simulink model "single_phase_afe_ideal"  (R2026a)
settings: Solver=ode23tb  StopTime=simlength  FixedStep=tc  MaxStep=glb_time.tc
values from neighbouring files (symbols this model uses):
  afe_ctrl = ctrl_afe_setup(glb_time.ts_afe, grid_emu.omega_grid_nom)    [init_model_legacy.m]
  frequency_set = 300    [init_model_legacy.m]
  glb_time = timing_setup(fpwm_afe, trgo_afe, fpwm_inv, trgo_inv, fpwm_single_phase_inv, trgo_single_phase_inv, fpwm_dab, trgo_dab,      fpwm_psfbc, trgo_psfbc, fpwm_isop_rail, trgo_isop_rail, fpwm_cllc, trgo_cllc, t_measure, tc_factor, tc_decimation, delay_pwm, dead_time_afe,      dead_time_inv, dead_time_single_phase_inv, dead_time_dab, dead_time_psfbc, dead_time_isop_rail, dead_time_cllc)    [init_model_legacy.m]
  grid_emu = grid_three_phase_emulator('Dyn11', delta_star, grid_nominal_power, application_voltage, us1, us2, fgrid,                  eq_grid_inductance, eq_grid_resistance, eta, ucc, i1m, p_iron, n1, n2, core_area, core_length, mur,                  up_xi_pu_ref, up_eta_pu_ref, un_xi_pu_ref, un_eta_pu_ref)    [init_model_legacy.m]
  heatsink = liquid_cooled_plate_2kw_setup(weight, no_weight, cp_al, heat_capacity_hs, thermal_conductivity_al,      Rth_switch_HA, Rth_mosfet_HA, Rth_diode_HA, Tambient, DThs_init)    [init_model_legacy.m]
  kepsilon = 2    [init_model_legacy.m]
  omega_set = frequency_set*2*pi    (= 1884.95559215)    [init_model_legacy.m]
  single_phase_inverter_ctrl = ctrl_single_phase_inverter_setup(glb_time.ts_inv, pres_ctrl.omega_set,      dqvector_pi.kp_inv, dqvector_pi.ki_inv, pres_ctrl.kp_rpi, pres_ctrl.ki_rpi, pres_ctrl.delta_rpi)    [init_model_legacy.m]
  Tambient = 40    [init_model_legacy.m]
  time_step_ref_1 = 0.025    [init_model_legacy.m]
  time_step_ref_2 = 0.5    [init_model_legacy.m]
  time_step_ref_3 = 1    [init_model_legacy.m]
  Vdc_nom = 400*1.35    (= 540)    [power_losses_calculation.m]
undefined symbols (not defined in the file or in its folder): delta_fht1, hwdata, igbt, Ld_fht1, magnitude, omega_fht1, ts_inv, Vac_FS, Xbez
libraries: fl_lib x116, nesl_utility x65, phase_shift_filter_ccaller x5, dq_vector_pi x4, igbt_simple_2th_lib x4, linear_double_integrator_observer_ccaller x3, lithium_ion_battery x1, dclink_for_two_levels x1, three_phase_voltage_with_frt_emulator x1, simulink x1, cstblocks_lti x1, single_phase_pwm_modulator x1
(part 4 of 6)

== system single_phase_afe_ideal/single_phase_inverter/single phase inverter control/single_phase_inverter_ctrl/phase generator/FHT-PLL/pll_stageA/filter_and_transformation ==
  ug_a : Inport
  ug_b : Inport  Port=2
  ug_c : Inport  Port=3
  Bus Creator : BusCreator  Inputs=2
  Bus Creator1 : BusCreator  Inputs=3
  Bus Creator2 : BusCreator  Inputs=2
  Bus Creator3 : BusCreator  Inputs=3
  Bus Creator4 : BusCreator  Inputs=3
  FHTalpha : Subsystem
  FHTbeta : Subsystem
  FHTdqPLL : Scope  NumInputPorts=2
      settings: ActiveDisplayYMinimum=-1.5258214459194912  ActiveDisplayYMaximum=1.5258228058860459  DataLoggingVariableName=ScopeData12
  Gain : Gain  Gain=-1/2
  Gain1 : Gain  Gain=-1/2
  Sum : Sum  Inputs=|++
  Sum1 : Sum  Inputs=-+|
  To Workspace1 : ToWorkspace  VariableName=ugd_alpha_sim  SampleTime=-1
      settings: MaxDataPoints=glb_time.Ns_afe
  To Workspace2 : ToWorkspace  VariableName=ugd_beta_sim  SampleTime=-1
      settings: MaxDataPoints=glb_time.Ns_afe
  To Workspace3 : ToWorkspace  VariableName=u_fht_alpha_sim  SampleTime=-1
      settings: MaxDataPoints=glb_time.Ns_afe
  To Workspace4 : ToWorkspace  VariableName=v_fht_alpha_sim  SampleTime=-1
      settings: MaxDataPoints=glb_time.Ns_afe
  To Workspace5 : ToWorkspace  VariableName=u_fhtsr_alpha_sim  SampleTime=-1
      settings: MaxDataPoints=glb_time.Ns_afe
  To Workspace6 : ToWorkspace  VariableName=u_fhtsr_beta_sim  SampleTime=-1
      settings: MaxDataPoints=glb_time.Ns_afe
  To Workspace7 : ToWorkspace  VariableName=u_fht_beta_sim  SampleTime=-1
      settings: MaxDataPoints=glb_time.Ns_afe
  To Workspace8 : ToWorkspace  VariableName=v_fht_beta_sim  SampleTime=-1
      settings: MaxDataPoints=glb_time.Ns_afe
  To Workspace9 : ToWorkspace  VariableName=ugd_abc_grid_sim  SampleTime=-1
      settings: MaxDataPoints=glb_time.Ns_afe
  abc2alphabeta : MATLAB Function  TreatAsAtomicUnit=on
  grid_voltages : Scope  NumInputPorts=3
      settings: ActiveDisplayYMinimum=-1.3620119839906693  ActiveDisplayYMaximum=1.3591613322496414  DataLoggingVariableName=ScopeData13
  ug_alpha : Outport  VectorParamsAs1DForOutWhenUnconnected=off
  ug_beta : Outport  Port=2  VectorParamsAs1DForOutWhenUnconnected=off
  wires:
  ug_b/1 -> Bus Creator3/2, grid_voltages/2, abc2alphabeta/2(b)  "ugd_b"
  ug_c/1 -> Bus Creator3/3, grid_voltages/3, abc2alphabeta/3(c)  "ugd_c"
  ug_a/1 -> Bus Creator3/1, grid_voltages/1, abc2alphabeta/1(a)  "ugd_a"
  abc2alphabeta/1(alpha) -> To Workspace1/1, FHTalpha/1(u), Bus Creator4/1  "u_grid_alpha"
  abc2alphabeta/2(beta) -> FHTbeta/1(u), To Workspace2/1, Bus Creator1/1  "u_grid_beta"
  FHTalpha/1(ud_hat) -> To Workspace3/1, Bus Creator/1, Sum/1  "u_fht_alpha"
  Sum/1 -> Gain/1
  FHTbeta/1(ud_hat) -> Sum1/2, To Workspace7/1, Bus Creator2/1  "u_fht_beta"
  Sum1/1 -> Gain1/1
  Gain1/1 -> Bus Creator1/3, To Workspace6/1, ug_beta/1  "u_fhtsr_beta"
  Gain/1 -> Bus Creator4/3, To Workspace5/1, ug_alpha/1  "u_fhtsr_alpha"
  FHTbeta/2(uq_hat) -> Sum/2, To Workspace8/1, Bus Creator2/2  "v_fht_beta"
  FHTalpha/2(uq_hat) -> Sum1/1, To Workspace4/1, Bus Creator/2  "v_fht_alpha"
  Bus Creator1/1 -> FHTdqPLL/2
  Bus Creator4/1 -> FHTdqPLL/1
  Bus Creator/1 -> Bus Creator4/2  "FHTalpha"
  Bus Creator2/1 -> Bus Creator1/2  "FHTbeta"
  Bus Creator3/1 -> To Workspace9/1

== system single_phase_afe_ideal/single_phase_inverter/single phase inverter control/single_phase_inverter_ctrl/phase generator/FHT-PLL/pll_stageA/sequences ==
  u_grid_alpha : Inport
  u_grid_beta : Inport  Port=2
  phase_angle : Inport  Port=3
  alphabeta2xieta : MATLAB Function  TreatAsAtomicUnit=on
  u_grid_xi : Outport
  u_grid_eta : Outport  Port=2
  wires:
  alphabeta2xieta/1(xi) -> u_grid_xi/1  "u_grid_xi"
  alphabeta2xieta/2(eta) -> u_grid_eta/1  "u_grid_eta"
  u_grid_alpha/1 -> alphabeta2xieta/1(alpha)  "u_grid_alpha"
  u_grid_beta/1 -> alphabeta2xieta/2(beta)  "u_grid_beta"
  phase_angle/1 -> alphabeta2xieta/3(gamma)  "phase_angle"

== system single_phase_afe_ideal/single_phase_inverter/single phase inverter control/single_phase_inverter_ctrl/phase generator/FHT-PLL/pll_stageB/double_integrator_observer ==
  theta : Inport
  Gain : Gain  Gain=afe_ctrl.di_obs.Ldso  Multiplication=Matrix(K*u)
  Gain1 : Gain  Gain=afe_ctrl.di_obs.Adso  Multiplication=Matrix(K*u)
  Gain2 : Gain  Gain=afe_ctrl.di_obs.Cso  Multiplication=Matrix(K*u)
  Selector : Selector  InputPortWidth=2  IndexOptions=Index vector (dialog)  Indices=2  OutputSizes=1
  Sum : Sum  Inputs=-+|
  Sum1 : Sum  Inputs=|++
  Unit Delay : UnitDelay  SampleTime=-1
  bounder1 : MATLAB Function  TreatAsAtomicUnit=on
  bounder2 : MATLAB Function  TreatAsAtomicUnit=on
  omega_hat : Outport
  wires:
  Gain/1 -> Sum1/1
  Selector/1 -> omega_hat/1
  Gain2/1 -> bounder2/1(u)  "theta_hat"
  Gain1/1 -> Sum1/2
  Sum1/1 -> Unit Delay/1
  Sum/1 -> bounder1/1(u)  "e"
  Unit Delay/1 -> Gain1/1, Selector/1, Gain2/1
  theta/1 -> Sum/2  "theta"
  bounder1/1(y) -> Gain/1
  bounder2/1(y) -> Sum/1  "theta_hat_bounded"

== system single_phase_afe_ideal/single_phase_inverter/single phase inverter control/single_phase_inverter_ctrl/single_phase_current_control/dqpi_current_controller/dq_vector_pi_ccaller/Reset ==
  Step : Step  Time=0.05  InitialValue=1  FinalValue=0
  en : Outport
  wires:
  Step/1 -> en/1

== system single_phase_afe_ideal/single_phase_inverter/single phase inverter control/single_phase_inverter_ctrl/single_phase_current_control/dqpi_current_controller/i2alphabeta/first_harmonic_tracker ==
  u : Inport
  Bus Selector : BusSelector  OutputSignals=output_pu_hat,output_pu_hat_dot
  Constant1 : Constant  Value=6
  Constant2 : Constant  Value=glb_time.ts_inv
  Constant3 : Constant  Value=afe_ctrl.fht_grid.omega_fht
  Constant4 : Constant  Value=afe_ctrl.fht_grid.delta_fht
  Constant5 : Constant  Value=afe_ctrl.fht_grid.Ld_fht(1)
  Constant6 : Constant  Value=afe_ctrl.fht_grid.Ld_fht(2)
  Data Type Conversion{1..2,6..9} (6 alike) : DataTypeConversion  OutDataTypeStr=single  SaturateOnIntegerOverflow=off  RndMeth=Floor
  Data Type Conversion10 : DataTypeConversion  OutDataTypeStr=double  SaturateOnIntegerOverflow=off  RndMeth=Floor
  Data Type Conversion3 : DataTypeConversion  OutDataTypeStr=uint8  SaturateOnIntegerOverflow=off  RndMeth=Floor
  Data Type Conversion4 : DataTypeConversion  OutDataTypeStr=double  SaturateOnIntegerOverflow=off  RndMeth=Floor
  Data Type Conversion5 : DataTypeConversion  OutDataTypeStr=uint8  SaturateOnIntegerOverflow=off  RndMeth=Floor
  Gain : Gain  Gain=-1/afe_ctrl.fht_grid.omega_fht
  Step : Step  Time=0.0125  InitialValue=1  FinalValue=0
  first_harmonic_tracker : CCaller  FunctionName=first_harmonic_tracker_process_simulink  PortSpecificationStruct="%)30     .    B \\   8    (     @         %    \"     D    !     0         %  0 \"0    $    _    07)G3F%M90  4&]R=$YA;64 4V-O<&4     26YD97@     5'EP90      4VEZ90      27-';&]B86P   X    P    !@    @    $          4    (     0    ,    !         !   P!O=70 #@   #     &    \"     0         !0    @    !     P    $         $  # &]U=  .    .     8    (    !          %    \"     $    &     0         0  ...(+4988 chars)"
  alpha : Outport
  beta : Outport  Port=2
  wires:
  Data Type Conversion4/1 -> alpha/1
  Data Type Conversion3/1 -> first_harmonic_tracker/1
  Data Type Conversion1/1 -> first_harmonic_tracker/3
  Data Type Conversion2/1 -> first_harmonic_tracker/2
  first_harmonic_tracker/1 -> Bus Selector/1
  Bus Selector/1 -> Data Type Conversion4/1  "<output_pu_hat>"
  Step/1 -> Data Type Conversion3/1
  u/1 -> Data Type Conversion2/1
  Constant2/1 -> Data Type Conversion1/1
  Constant1/1 -> Data Type Conversion5/1
  Data Type Conversion5/1 -> first_harmonic_tracker/8
  Constant3/1 -> Data Type Conversion6/1
  Data Type Conversion6/1 -> first_harmonic_tracker/4
  Constant4/1 -> Data Type Conversion7/1
  Data Type Conversion7/1 -> first_harmonic_tracker/5
  Constant5/1 -> Data Type Conversion8/1
  Data Type Conversion8/1 -> first_harmonic_tracker/6
  Constant6/1 -> Data Type Conversion9/1
  Data Type Conversion9/1 -> first_harmonic_tracker/7
  Bus Selector/2 -> Data Type Conversion10/1  "<output_pu_hat_dot>"
  Data Type Conversion10/1 -> Gain/1
  Gain/1 -> beta/1

== system single_phase_afe_ideal/single_phase_inverter/single phase inverter control/single_phase_inverter_ctrl/single_phase_current_control/dqpi_current_controller/i2alphabeta/phase_shift_method ==
  i_alpha : Inport
  Gain : Gain  Gain=-1
  phase shift filter : phase_shift_filter/phase shift filter  f=frequency_set  scaling_factor=1  ts=glb_time.ts_inv
  i_alpha_phase_shift_m : Outport
  i_beta_phase_shift_m : Outport  Port=2
  wires:
  i_alpha/1 -> phase shift filter/1, i_alpha_phase_shift_m/1
  Gain/1 -> i_beta_phase_shift_m/1  "i_beta_phase_shift_methos"
  phase shift filter/1 -> Gain/1

== system single_phase_afe_ideal/single_phase_inverter/single phase inverter control/single_phase_inverter_ctrl/single_phase_current_control/dqpi_current_controller/i2alphabeta/phase_shift_method_ccaller ==
  i_alpha : Inport
  Gain : Gain  Gain=-1
  phase_shift_filter_ccaller : phase_shift_filter_ccaller/phase_shift_filter_ccaller  freq_m=frequency_set  ts_m=glb_time.ts_inv  scaling_m=1  reset_time_release=0.025  instance=0  tc_m=-1
  i_alpha_phase_shift_m : Outport
  i_beta_phase_shift_m : Outport  Port=2
  wires:
  phase_shift_filter_ccaller/1 -> Gain/1
  Gain/1 -> i_beta_phase_shift_m/1  "i_beta_phase_shift_methos"
  i_alpha/1 -> i_alpha_phase_shift_m/1, phase_shift_filter_ccaller/1

== system single_phase_afe_ideal/single_phase_inverter/single phase inverter control/single_phase_inverter_ctrl/single_phase_current_control/dqpi_current_controller/i2alphabeta/sogi ==
  u : Inport
  Constant2 : Constant  Value=omega_set
  Product : Product
  Product1 : Product
  Sum1 : Sum  Inputs=|+-
  Sum3 : Sum  Inputs=-+|
  integrator_1 : Subsystem
  integrator_2 : Subsystem
  kepsilon : Gain  Gain=kepsilon
  ualpha : Outport
  ubeta : Outport  Port=2
  wires:
  u/1 -> ualpha/1, Sum3/2
  Sum3/1 -> kepsilon/1
  kepsilon/1 -> Sum1/1
  Sum1/1 -> Product/2
  Product/1 -> integrator_1/1(in)
  integrator_1/1(out) -> Product1/2, Sum3/1
  Constant2/1 -> Product/1, Product1/1
  Product1/1 -> integrator_2/1(in)
  integrator_2/1(out) -> ubeta/1, Sum1/2

== system single_phase_afe_ideal/single_phase_inverter/single phase inverter control/single_phase_inverter_ctrl/single_phase_current_control/dqpi_current_controller/i2alphabeta/sogi_ccaller ==
  input : Inport
  Bus Selector : BusSelector  OutputSignals=sogi_flt_output_alpha,sogi_flt_output_beta
  CCaller : CCaller  FunctionName=sogi_flt_process_simulink  PortSpecificationStruct="%)30     .    . P   8    (     @         %    \"     <    !     0         %  0 \"0    $    _    07)G3F%M90  4&]R=$YA;64 4V-O<&4     26YD97@     5'EP90      4VEZ90      27-';&]B86P   X    P    !@    @    $          4    (     0    ,    !         !   P!O=70 #@   #     &    \"     0         !0    @    !     P    $         $  # &]U=  .    .     8    (    !          %    \"     $    &     0         0   ...(+3829 chars)"
  Constant1 : Constant  Value=glb_time.ts_inv
  Constant2 : Constant  Value=omega_set
  Constant3 : Constant  Value=kepsilon
  Constant4 : Constant  Value=2
  Data Type Conversion{1..2,4,6} (4 alike) : DataTypeConversion  OutDataTypeStr=single  SaturateOnIntegerOverflow=off  RndMeth=Floor
  Data Type Conversion3 : DataTypeConversion  OutDataTypeStr=uint8  SaturateOnIntegerOverflow=off  RndMeth=Floor
  Data Type Conversion5 : DataTypeConversion  OutDataTypeStr=double  SaturateOnIntegerOverflow=off  RndMeth=Floor
  Data Type Conversion7 : DataTypeConversion  OutDataTypeStr=double  SaturateOnIntegerOverflow=off  RndMeth=Floor
  Data Type Conversion8 : DataTypeConversion  OutDataTypeStr=uint8  SaturateOnIntegerOverflow=off  RndMeth=Floor
  Reset : Subsystem
  Terminator : Terminator
  Zero-Order Hold{1..6} (6 alike) : ZeroOrderHold  SampleTime=-1
  alpha : Outport
  beta : Outport  Port=2
  wires:
  Zero-Order Hold6/1 -> Data Type Conversion4/1
  Data Type Conversion4/1 -> CCaller/1
  Bus Selector/1 -> Data Type Conversion7/1  "<sogi_flt_output_alpha>"
  CCaller/1 -> Bus Selector/1
  Constant4/1 -> Zero-Order Hold5/1
  Zero-Order Hold5/1 -> Data Type Conversion3/1
  Constant2/1 -> Zero-Order Hold1/1
  Zero-Order Hold1/1 -> Data Type Conversion2/1
  Zero-Order Hold2/1 -> Data Type Conversion1/1
  Constant1/1 -> Zero-Order Hold2/1
  Reset/1(en) -> Zero-Order Hold4/1
  Zero-Order Hold4/1 -> Data Type Conversion8/1
  input/1 -> alpha/1, Zero-Order Hold6/1
  Bus Selector/2 -> Data Type Conversion5/1  "<sogi_flt_output_beta>"
  Data Type Conversion5/1 -> beta/1
  Data Type Conversion3/1 -> CCaller/6
  Data Type Conversion8/1 -> CCaller/5
  Data Type Conversion2/1 -> CCaller/3
  Data Type Conversion1/1 -> CCaller/2
  Data Type Conversion6/1 -> CCaller/4
  Zero-Order Hold3/1 -> Data Type Conversion6/1
  Constant3/1 -> Zero-Order Hold3/1
  Data Type Conversion7/1 -> Terminator/1

== system single_phase_afe_ideal/single_phase_inverter/single phase inverter control/single_phase_inverter_ctrl/sistem_identification/open loop u//f/sogi_ccaller/Reset ==
  Step : Step  Time=0.025  InitialValue=1  FinalValue=0
  en : Outport
  wires:
  Step/1 -> en/1

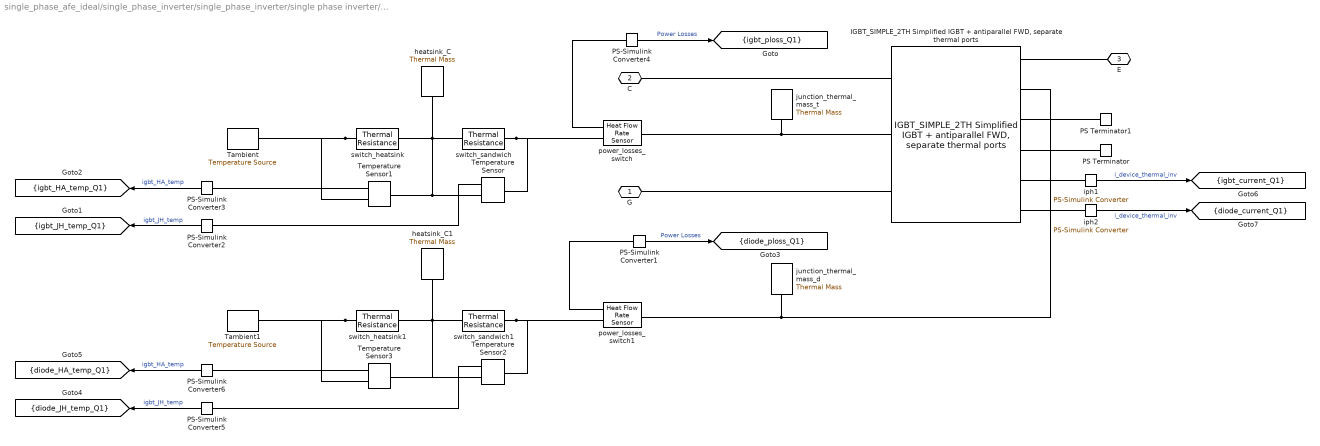
== system single_phase_afe_ideal/single_phase_inverter/single_phase_inverter/single phase inverter/three_phase_inverter_with_igbt_simple_2th/full_bridge_with_igbt_simple_2th/igbt_simple_1/IGBT_simple ==
  "IGBT_SIMPLE_2TH Simplified IGBT + antiparallel FWD, separate thermal ports" : igbt_simple_2th_lib/IGBT_SIMPLE_2TH Simplified IGBT + antiparallel FWD, separate thermal ports  Vce_sat=vce_sat_m V  Vf=v_gamma_m V  Vth=Vth_gate_m V  Vhyst=Vth_gate_hyst_m V  Eon_ref=Eon_m mJ  Eoff_ref=Eoff_m mJ  Err_ref=Err_m mJ  Ic_ref=Ic_ref_m A  Vdc_ref=Vdc_ref_m V  V_rr_th=Vblock_Errf_m V  Ron=rce_on_m mOhm  Rd=rd_on_m mOhm  Goff=Gce_off_m 1/Ohm  tau_s=time_constant_edge_m us  tau_p=time_constant_ploss_m us  i_specify=off  i_priority=None  i=0 A  i_nominal_specify=off  i_nominal_value=1  i_nominal_unit=A  v_specify=off  v_priority=None  v=0 V  v_nominal_specify=off  v_nominal_value=1  v_nominal_unit=V  i_t_specify=off  i_t_priority=None  i_t=0 A  i_t_nominal_specify=off  i_t_nominal_value=1  i_t_nominal_unit=A  i_d_specify=off  i_d_priority=None  i_d=0 A  i_d_nominal_specify=off  i_d_nominal_value=1  i_d_nominal_unit=A  i_h_specify=off  i_h_priority=None  i_h=0 A  i_h_nominal_specify=off  i_h_nominal_value=1  i_h_nominal_unit=A  i_dh_specify=off  i_dh_priority=None  i_dh=0 A  i_dh_nominal_specify=off  i_dh_nominal_value=1  i_dh_nominal_unit=A  v_h_specify=off  v_h_priority=None  v_h=0 V  v_h_nominal_specify=off  v_h_nominal_value=1  v_h_nominal_unit=V  E_lpt_specify=off  E_lpt_priority=None  E_lpt=0 J  E_lpt_nominal_specify=off  E_lpt_nominal_value=1  E_lpt_nominal_unit=J  E_lpd_specify=off  E_lpd_priority=None  E_lpd=0 J  E_lpd_nominal_specify=off  E_lpd_nominal_value=1  E_lpd_nominal_unit=J  Qt_specify=off  Qt_priority=None  Qt=0 W  Qt_nominal_specify=off  Qt_nominal_value=1  Qt_nominal_unit=W  Qd_specify=off  Qd_priority=None  Qd=0 W  Qd_nominal_specify=off  Qd_nominal_value=1  Qd_nominal_unit=W  E_t_specify=off  E_t_priority=None  E_t=0 J  E_d_specify=off  E_d_priority=None  E_d=0 J
  PS Terminator : fl_lib/Physical Signals/Sinks/PS Terminator
  PS Terminator1 : fl_lib/Physical Signals/Sinks/PS Terminator
  PS-Simulink Converter1 : nesl_utility/PS-Simulink Converter  PhysicalDomain=network_engine_domain  SubClassName=ps_output  LeftPortType=input  RightPortType=output  PseudoPeriodic=off  Frequencies=[]  VectorFormat=1-D array  Unit=J/s  AffineConversion=off
  PS-Simulink Converter{2..3,5..6} (4 alike) : nesl_utility/PS-Simulink Converter  PhysicalDomain=network_engine_domain  SubClassName=ps_output  LeftPortType=input  RightPortType=output  PseudoPeriodic=off  Frequencies=[]  VectorFormat=1-D array  Unit=degC  AffineConversion=off
  PS-Simulink Converter4 : nesl_utility/PS-Simulink Converter  PhysicalDomain=network_engine_domain  SubClassName=ps_output  LeftPortType=input  RightPortType=output  PseudoPeriodic=off  Frequencies=[]  VectorFormat=1-D array  Unit=J/s  AffineConversion=off
  Tambient : fl_lib/Thermal/Thermal Sources/Temperature Source  temperature=Tambient_m degC
  Tambient1 : fl_lib/Thermal/Thermal Sources/Temperature Source  temperature=Tambient_m degC
  Temperature Sensor{,1..3} (4 alike) : fl_lib/Thermal/Thermal Sensors/Temperature Sensor  temperature_measure=foundation.enum.MeasurementReference.difference
  heatsink_C : fl_lib/Thermal/Thermal Elements/Thermal Mass  mass_type=foundation.enum.constant_variable.constant  mass=mass_heatsink_m kg  sp_heat=specific_heat_m J/(K*kg)  mass_min=1e-6 kg  num_ports=foundation.enum.numPorts2.one  m_specify=off  m_priority=High  m=1 kg  m_nominal_specify=off  m_nominal_value=1  m_nominal_unit=kg  T_specify=on  T_priority=High  T=Tambient_m degC  T_nominal_specify=off  T_nominal_value=1  T_nominal_unit=K  Q_specify=off  Q_priority=High  Q=0 W  Q_nominal_specify=off  Q_nominal_value=1  Q_nominal_unit=W
  heatsink_C1 : fl_lib/Thermal/Thermal Elements/Thermal Mass  mass_type=foundation.enum.constant_variable.constant  mass=mass_heatsink_m kg  sp_heat=specific_heat_m J/(K*kg)  mass_min=1e-6 kg  num_ports=foundation.enum.numPorts2.one  m_specify=off  m_priority=High  m=1 kg  m_nominal_specify=off  m_nominal_value=1  m_nominal_unit=kg  T_specify=on  T_priority=High  T=Tambient_m degC  T_nominal_specify=off  T_nominal_value=1  T_nominal_unit=K  Q_specify=off  Q_priority=High  Q=0 W  Q_nominal_specify=off  Q_nominal_value=1  Q_nominal_unit=W
  iph1 : nesl_utility/PS-Simulink Converter  PhysicalDomain=network_engine_domain  SubClassName=ps_output  LeftPortType=input  RightPortType=output  PseudoPeriodic=off  Frequencies=[]  VectorFormat=1-D array  Unit=A  AffineConversion=off
  iph2 : nesl_utility/PS-Simulink Converter  PhysicalDomain=network_engine_domain  SubClassName=ps_output  LeftPortType=input  RightPortType=output  PseudoPeriodic=off  Frequencies=[]  VectorFormat=1-D array  Unit=A  AffineConversion=off
  junction_thermal_mass_d : fl_lib/Thermal/Thermal Elements/Thermal Mass  mass_type=foundation.enum.constant_variable.constant  mass=JunctionTermalMass_m/specific_heat_m kg  sp_heat=specific_heat_m J/(K*kg)  mass_min=1e-6 kg  num_ports=foundation.enum.numPorts2.one  m_specify=off  m_priority=High  m=1 kg  m_nominal_specify=off  m_nominal_value=1  m_nominal_unit=kg  T_specify=on  T_priority=High  T=Tambient_m degC  T_nominal_specify=off  T_nominal_value=1  T_nominal_unit=K  Q_specify=off  Q_priority=High  Q=0 W  Q_nominal_specify=off  Q_nominal_value=1  Q_nominal_unit=W
  junction_thermal_mass_t : fl_lib/Thermal/Thermal Elements/Thermal Mass  mass_type=foundation.enum.constant_variable.constant  mass=JunctionTermalMass_m/specific_heat_m kg  sp_heat=specific_heat_m J/(K*kg)  mass_min=1e-6 kg  num_ports=foundation.enum.numPorts2.one  m_specify=off  m_priority=High  m=1 kg  m_nominal_specify=off  m_nominal_value=1  m_nominal_unit=kg  T_specify=on  T_priority=High  T=Tambient_m degC  T_nominal_specify=off  T_nominal_value=1  T_nominal_unit=K  Q_specify=off  Q_priority=High  Q=0 W  Q_nominal_specify=off  Q_nominal_value=1  Q_nominal_unit=W
  power_losses_switch : fl_lib/Thermal/Thermal Sensors/Heat Flow Rate Sensor
  power_losses_switch1 : fl_lib/Thermal/Thermal Sensors/Heat Flow Rate Sensor
  switch_heatsink : fl_lib/Thermal/Thermal Elements/Thermal Resistance  resistance=rth_switch_HA_m K/W  T_specify=off  T_priority=High  T=0 deltadegC  T_nominal_specify=off  T_nominal_value=1  T_nominal_unit=K  Q_specify=off  Q_priority=None  Q=0 W  Q_nominal_specify=off  Q_nominal_value=1  Q_nominal_unit=W
  switch_heatsink1 : fl_lib/Thermal/Thermal Elements/Thermal Resistance  resistance=rth_diode_HA_m K/W  T_specify=off  T_priority=High  T=0 deltadegC  T_nominal_specify=off  T_nominal_value=1  T_nominal_unit=K  Q_specify=off  Q_priority=None  Q=0 W  Q_nominal_specify=off  Q_nominal_value=1  Q_nominal_unit=W
  switch_sandwich : fl_lib/Thermal/Thermal Elements/Thermal Resistance  resistance=rth_switch_JH_m K/W  T_specify=off  T_priority=High  T=0 degC  T_nominal_specify=off  T_nominal_value=1  T_nominal_unit=K  Q_specify=off  Q_priority=None  Q=0 W  Q_nominal_specify=off  Q_nominal_value=1  Q_nominal_unit=W
  switch_sandwich1 : fl_lib/Thermal/Thermal Elements/Thermal Resistance  resistance=rth_diode_JH_m K/W  T_specify=off  T_priority=High  T=0 degC  T_nominal_specify=off  T_nominal_value=1  T_nominal_unit=K  Q_specify=off  Q_priority=None  Q=0 W  Q_nominal_specify=off  Q_nominal_value=1  Q_nominal_unit=W
  G : PMIOPort  Side=Left
  C : PMIOPort  Port=2  Side=Left
  E : PMIOPort  Port=3  Side=Right
  tag scope: diode_HA_temp_Q1=scoped, diode_JH_temp_Q1=scoped, diode_current_Q1=scoped, diode_ploss_Q1=scoped, igbt_HA_temp_Q1=scoped, igbt_JH_temp_Q1=scoped, igbt_current_Q1=scoped, igbt_ploss_Q1=scoped
  wires:
  PS-Simulink Converter3/1 -> [igbt_HA_temp_Q1]  "igbt_HA_temp"
  PS-Simulink Converter4/1 -> [igbt_ploss_Q1]  "Power Losses"
  PS-Simulink Converter2/1 -> [igbt_JH_temp_Q1]  "igbt_JH_temp"
  PS-Simulink Converter1/1 -> [diode_ploss_Q1]  "Power Losses"
  PS-Simulink Converter5/1 -> [diode_JH_temp_Q1]  "igbt_JH_temp"
  PS-Simulink Converter6/1 -> [diode_HA_temp_Q1]  "igbt_HA_temp"
  iph1/1 -> [igbt_current_Q1]  "i_device_thermal_inv"
  iph2/1 -> [diode_current_Q1]  "i_device_thermal_inv"
  connections:
  Temperature Sensor/RConn2 -- PS-Simulink Converter2/LConn1
  "IGBT_SIMPLE_2TH Simplified IGBT + antiparallel FWD, separate thermal ports"/LConn2 -- junction_thermal_mass_t/LConn1 -- power_losses_switch/LConn1
  Temperature Sensor1/RConn2 -- PS-Simulink Converter3/LConn1
  Temperature Sensor1/LConn1 -- Temperature Sensor/RConn1 -- switch_heatsink/LConn1 -- heatsink_C/LConn1 -- switch_sandwich/RConn1
  switch_heatsink/RConn1 -- Tambient/LConn1 -- Temperature Sensor1/RConn1
  switch_sandwich/LConn1 -- power_losses_switch/RConn2 -- Temperature Sensor/LConn1
  "IGBT_SIMPLE_2TH Simplified IGBT + antiparallel FWD, separate thermal ports"/RConn1 -- E/RConn1
  "IGBT_SIMPLE_2TH Simplified IGBT + antiparallel FWD, separate thermal ports"/LConn1 -- C/RConn1
  "IGBT_SIMPLE_2TH Simplified IGBT + antiparallel FWD, separate thermal ports"/LConn3 -- G/RConn1
  switch_heatsink1/LConn1 -- switch_sandwich1/RConn1 -- heatsink_C1/LConn1 -- Temperature Sensor2/RConn1 -- Temperature Sensor3/LConn1
  switch_heatsink1/RConn1 -- Temperature Sensor3/RConn1 -- Tambient1/LConn1
  switch_sandwich1/LConn1 -- Temperature Sensor2/LConn1 -- power_losses_switch1/RConn2
  Temperature Sensor3/RConn2 -- PS-Simulink Converter6/LConn1
  Temperature Sensor2/RConn2 -- PS-Simulink Converter5/LConn1
  power_losses_switch1/LConn1 -- "IGBT_SIMPLE_2TH Simplified IGBT + antiparallel FWD, separate thermal ports"/RConn2 -- junction_thermal_mass_d/LConn1
  "IGBT_SIMPLE_2TH Simplified IGBT + antiparallel FWD, separate thermal ports"/RConn5 -- iph1/LConn1
  "IGBT_SIMPLE_2TH Simplified IGBT + antiparallel FWD, separate thermal ports"/RConn6 -- iph2/LConn1
  PS Terminator1/LConn1 -- "IGBT_SIMPLE_2TH Simplified IGBT + antiparallel FWD, separate thermal ports"/RConn3
  PS Terminator/LConn1 -- "IGBT_SIMPLE_2TH Simplified IGBT + antiparallel FWD, separate thermal ports"/RConn4
  PS-Simulink Converter4/LConn1 -- power_losses_switch/RConn1
  PS-Simulink Converter1/LConn1 -- power_losses_switch1/RConn1

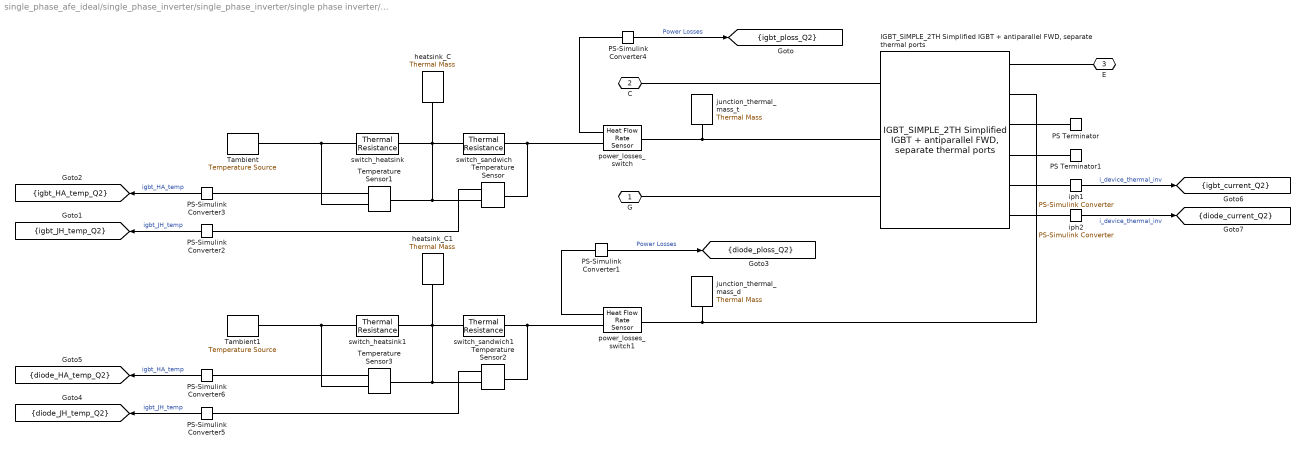
== system single_phase_afe_ideal/single_phase_inverter/single_phase_inverter/single phase inverter/three_phase_inverter_with_igbt_simple_2th/full_bridge_with_igbt_simple_2th/igbt_simple_2/IGBT_simple ==
  "IGBT_SIMPLE_2TH Simplified IGBT + antiparallel FWD, separate thermal ports" : igbt_simple_2th_lib/IGBT_SIMPLE_2TH Simplified IGBT + antiparallel FWD, separate thermal ports  Vce_sat=vce_sat_m V  Vf=v_gamma_m V  Vth=Vth_gate_m V  Vhyst=Vth_gate_hyst_m V  Eon_ref=Eon_m mJ  Eoff_ref=Eoff_m mJ  Err_ref=Err_m mJ  Ic_ref=Ic_ref_m A  Vdc_ref=Vdc_ref_m V  V_rr_th=Vblock_Errf_m V  Ron=rce_on_m mOhm  Rd=rd_on_m mOhm  Goff=Gce_off_m 1/Ohm  tau_s=time_constant_edge_m us  tau_p=time_constant_ploss_m us  i_specify=off  i_priority=None  i=0 A  i_nominal_specify=off  i_nominal_value=1  i_nominal_unit=A  v_specify=off  v_priority=None  v=0 V  v_nominal_specify=off  v_nominal_value=1  v_nominal_unit=V  i_t_specify=off  i_t_priority=None  i_t=0 A  i_t_nominal_specify=off  i_t_nominal_value=1  i_t_nominal_unit=A  i_d_specify=off  i_d_priority=None  i_d=0 A  i_d_nominal_specify=off  i_d_nominal_value=1  i_d_nominal_unit=A  i_h_specify=off  i_h_priority=None  i_h=0 A  i_h_nominal_specify=off  i_h_nominal_value=1  i_h_nominal_unit=A  i_dh_specify=off  i_dh_priority=None  i_dh=0 A  i_dh_nominal_specify=off  i_dh_nominal_value=1  i_dh_nominal_unit=A  v_h_specify=off  v_h_priority=None  v_h=0 V  v_h_nominal_specify=off  v_h_nominal_value=1  v_h_nominal_unit=V  E_lpt_specify=off  E_lpt_priority=None  E_lpt=0 J  E_lpt_nominal_specify=off  E_lpt_nominal_value=1  E_lpt_nominal_unit=J  E_lpd_specify=off  E_lpd_priority=None  E_lpd=0 J  E_lpd_nominal_specify=off  E_lpd_nominal_value=1  E_lpd_nominal_unit=J  Qt_specify=off  Qt_priority=None  Qt=0 W  Qt_nominal_specify=off  Qt_nominal_value=1  Qt_nominal_unit=W  Qd_specify=off  Qd_priority=None  Qd=0 W  Qd_nominal_specify=off  Qd_nominal_value=1  Qd_nominal_unit=W  E_t_specify=off  E_t_priority=None  E_t=0 J  E_d_specify=off  E_d_priority=None  E_d=0 J
  PS Terminator : fl_lib/Physical Signals/Sinks/PS Terminator
  PS Terminator1 : fl_lib/Physical Signals/Sinks/PS Terminator
  PS-Simulink Converter1 : nesl_utility/PS-Simulink Converter  PhysicalDomain=network_engine_domain  SubClassName=ps_output  LeftPortType=input  RightPortType=output  PseudoPeriodic=off  Frequencies=[]  VectorFormat=1-D array  Unit=J/s  AffineConversion=off
  PS-Simulink Converter{2..3,5..6} (4 alike) : nesl_utility/PS-Simulink Converter  PhysicalDomain=network_engine_domain  SubClassName=ps_output  LeftPortType=input  RightPortType=output  PseudoPeriodic=off  Frequencies=[]  VectorFormat=1-D array  Unit=degC  AffineConversion=off
  PS-Simulink Converter4 : nesl_utility/PS-Simulink Converter  PhysicalDomain=network_engine_domain  SubClassName=ps_output  LeftPortType=input  RightPortType=output  PseudoPeriodic=off  Frequencies=[]  VectorFormat=1-D array  Unit=J/s  AffineConversion=off
  Tambient : fl_lib/Thermal/Thermal Sources/Temperature Source  temperature=Tambient_m degC
  Tambient1 : fl_lib/Thermal/Thermal Sources/Temperature Source  temperature=Tambient_m degC
  Temperature Sensor{,1..3} (4 alike) : fl_lib/Thermal/Thermal Sensors/Temperature Sensor  temperature_measure=foundation.enum.MeasurementReference.difference
  heatsink_C : fl_lib/Thermal/Thermal Elements/Thermal Mass  mass_type=foundation.enum.constant_variable.constant  mass=mass_heatsink_m kg  sp_heat=specific_heat_m J/(K*kg)  mass_min=1e-6 kg  num_ports=foundation.enum.numPorts2.one  m_specify=off  m_priority=High  m=1 kg  m_nominal_specify=off  m_nominal_value=1  m_nominal_unit=kg  T_specify=on  T_priority=High  T=Tambient_m degC  T_nominal_specify=off  T_nominal_value=1  T_nominal_unit=K  Q_specify=off  Q_priority=High  Q=0 W  Q_nominal_specify=off  Q_nominal_value=1  Q_nominal_unit=W
  heatsink_C1 : fl_lib/Thermal/Thermal Elements/Thermal Mass  mass_type=foundation.enum.constant_variable.constant  mass=mass_heatsink_m kg  sp_heat=specific_heat_m J/(K*kg)  mass_min=1e-6 kg  num_ports=foundation.enum.numPorts2.one  m_specify=off  m_priority=High  m=1 kg  m_nominal_specify=off  m_nominal_value=1  m_nominal_unit=kg  T_specify=on  T_priority=High  T=Tambient_m degC  T_nominal_specify=off  T_nominal_value=1  T_nominal_unit=K  Q_specify=off  Q_priority=High  Q=0 W  Q_nominal_specify=off  Q_nominal_value=1  Q_nominal_unit=W
  iph1 : nesl_utility/PS-Simulink Converter  PhysicalDomain=network_engine_domain  SubClassName=ps_output  LeftPortType=input  RightPortType=output  PseudoPeriodic=off  Frequencies=[]  VectorFormat=1-D array  Unit=A  AffineConversion=off
  iph2 : nesl_utility/PS-Simulink Converter  PhysicalDomain=network_engine_domain  SubClassName=ps_output  LeftPortType=input  RightPortType=output  PseudoPeriodic=off  Frequencies=[]  VectorFormat=1-D array  Unit=A  AffineConversion=off
  junction_thermal_mass_d : fl_lib/Thermal/Thermal Elements/Thermal Mass  mass_type=foundation.enum.constant_variable.constant  mass=JunctionTermalMass_m/specific_heat_m kg  sp_heat=specific_heat_m J/(K*kg)  mass_min=1e-6 kg  num_ports=foundation.enum.numPorts2.one  m_specify=off  m_priority=High  m=1 kg  m_nominal_specify=off  m_nominal_value=1  m_nominal_unit=kg  T_specify=on  T_priority=High  T=Tambient_m degC  T_nominal_specify=off  T_nominal_value=1  T_nominal_unit=K  Q_specify=off  Q_priority=High  Q=0 W  Q_nominal_specify=off  Q_nominal_value=1  Q_nominal_unit=W
  junction_thermal_mass_t : fl_lib/Thermal/Thermal Elements/Thermal Mass  mass_type=foundation.enum.constant_variable.constant  mass=JunctionTermalMass_m/specific_heat_m kg  sp_heat=specific_heat_m J/(K*kg)  mass_min=1e-6 kg  num_ports=foundation.enum.numPorts2.one  m_specify=off  m_priority=High  m=1 kg  m_nominal_specify=off  m_nominal_value=1  m_nominal_unit=kg  T_specify=on  T_priority=High  T=Tambient_m degC  T_nominal_specify=off  T_nominal_value=1  T_nominal_unit=K  Q_specify=off  Q_priority=High  Q=0 W  Q_nominal_specify=off  Q_nominal_value=1  Q_nominal_unit=W
  power_losses_switch : fl_lib/Thermal/Thermal Sensors/Heat Flow Rate Sensor
  power_losses_switch1 : fl_lib/Thermal/Thermal Sensors/Heat Flow Rate Sensor
  switch_heatsink : fl_lib/Thermal/Thermal Elements/Thermal Resistance  resistance=rth_switch_HA_m K/W  T_specify=off  T_priority=High  T=0 deltadegC  T_nominal_specify=off  T_nominal_value=1  T_nominal_unit=K  Q_specify=off  Q_priority=None  Q=0 W  Q_nominal_specify=off  Q_nominal_value=1  Q_nominal_unit=W
  switch_heatsink1 : fl_lib/Thermal/Thermal Elements/Thermal Resistance  resistance=rth_diode_HA_m K/W  T_specify=off  T_priority=High  T=0 deltadegC  T_nominal_specify=off  T_nominal_value=1  T_nominal_unit=K  Q_specify=off  Q_priority=None  Q=0 W  Q_nominal_specify=off  Q_nominal_value=1  Q_nominal_unit=W
  switch_sandwich : fl_lib/Thermal/Thermal Elements/Thermal Resistance  resistance=rth_switch_JH_m K/W  T_specify=off  T_priority=High  T=0 degC  T_nominal_specify=off  T_nominal_value=1  T_nominal_unit=K  Q_specify=off  Q_priority=None  Q=0 W  Q_nominal_specify=off  Q_nominal_value=1  Q_nominal_unit=W
  switch_sandwich1 : fl_lib/Thermal/Thermal Elements/Thermal Resistance  resistance=rth_diode_JH_m K/W  T_specify=off  T_priority=High  T=0 degC  T_nominal_specify=off  T_nominal_value=1  T_nominal_unit=K  Q_specify=off  Q_priority=None  Q=0 W  Q_nominal_specify=off  Q_nominal_value=1  Q_nominal_unit=W
  G : PMIOPort  Side=Left
  C : PMIOPort  Port=2  Side=Left
  E : PMIOPort  Port=3  Side=Right
  tag scope: diode_HA_temp_Q2=scoped, diode_JH_temp_Q2=scoped, diode_current_Q2=scoped, diode_ploss_Q2=scoped, igbt_HA_temp_Q2=scoped, igbt_JH_temp_Q2=scoped, igbt_current_Q2=scoped, igbt_ploss_Q2=scoped
  wires:
  iph2/1 -> [diode_current_Q2]  "i_device_thermal_inv"
  iph1/1 -> [igbt_current_Q2]  "i_device_thermal_inv"
  PS-Simulink Converter6/1 -> [diode_HA_temp_Q2]  "igbt_HA_temp"
  PS-Simulink Converter5/1 -> [diode_JH_temp_Q2]  "igbt_JH_temp"
  PS-Simulink Converter1/1 -> [diode_ploss_Q2]  "Power Losses"
  PS-Simulink Converter2/1 -> [igbt_JH_temp_Q2]  "igbt_JH_temp"
  PS-Simulink Converter4/1 -> [igbt_ploss_Q2]  "Power Losses"
  PS-Simulink Converter3/1 -> [igbt_HA_temp_Q2]  "igbt_HA_temp"
  connections:
  iph2/LConn1 -- "IGBT_SIMPLE_2TH Simplified IGBT + antiparallel FWD, separate thermal ports"/RConn6
  iph1/LConn1 -- "IGBT_SIMPLE_2TH Simplified IGBT + antiparallel FWD, separate thermal ports"/RConn5
  power_losses_switch1/LConn1 -- junction_thermal_mass_d/LConn1 -- "IGBT_SIMPLE_2TH Simplified IGBT + antiparallel FWD, separate thermal ports"/RConn2
  Temperature Sensor2/RConn2 -- PS-Simulink Converter5/LConn1
  Temperature Sensor3/RConn2 -- PS-Simulink Converter6/LConn1
  Temperature Sensor2/LConn1 -- switch_sandwich1/LConn1 -- power_losses_switch1/RConn2
  Temperature Sensor3/RConn1 -- switch_heatsink1/RConn1 -- Tambient1/LConn1
  Temperature Sensor3/LConn1 -- Temperature Sensor2/RConn1 -- switch_sandwich1/RConn1 -- switch_heatsink1/LConn1 -- heatsink_C1/LConn1
  "IGBT_SIMPLE_2TH Simplified IGBT + antiparallel FWD, separate thermal ports"/LConn3 -- G/RConn1
  "IGBT_SIMPLE_2TH Simplified IGBT + antiparallel FWD, separate thermal ports"/LConn1 -- C/RConn1
  "IGBT_SIMPLE_2TH Simplified IGBT + antiparallel FWD, separate thermal ports"/RConn1 -- E/RConn1
  Temperature Sensor/LConn1 -- power_losses_switch/RConn2 -- switch_sandwich/LConn1
  Temperature Sensor1/RConn1 -- Tambient/LConn1 -- switch_heatsink/RConn1
  Temperature Sensor/RConn1 -- Temperature Sensor1/LConn1 -- switch_sandwich/RConn1 -- heatsink_C/LConn1 -- switch_heatsink/LConn1
  Temperature Sensor1/RConn2 -- PS-Simulink Converter3/LConn1
  "IGBT_SIMPLE_2TH Simplified IGBT + antiparallel FWD, separate thermal ports"/LConn2 -- junction_thermal_mass_t/LConn1 -- power_losses_switch/LConn1
  Temperature Sensor/RConn2 -- PS-Simulink Converter2/LConn1
  PS Terminator1/LConn1 -- "IGBT_SIMPLE_2TH Simplified IGBT + antiparallel FWD, separate thermal ports"/RConn4
  PS Terminator/LConn1 -- "IGBT_SIMPLE_2TH Simplified IGBT + antiparallel FWD, separate thermal ports"/RConn3
  PS-Simulink Converter4/LConn1 -- power_losses_switch/RConn1
  PS-Simulink Converter1/LConn1 -- power_losses_switch1/RConn1
